simulink model "Porsche930Turbo_Model_V0"  (R2025b)
settings: Solver=ode3  StartTime=0.0  StopTime=1800  FixedStep=0.005  MaxStep=0.01  RelTol=1e-3
values from neighbouring files (symbols this model uses):
  a_front = (1 - CoG_front) * wb    (= 1.32912)    [Main.m]
  af = 1.77    [Main.m]
  bsfc = 395    [Main.m]
  cd = 0.39    [Main.m]
  crr = 0.015    [Main.m]
  distance_imola = s_track    [Main.m]
  eta_gb = 0.95    [Main.m]
  gear_numbers = [1, 2, 3, 4]    [Main.m]
  gear_ratios = [2.25, 1.30, 0.89, 0.625]    [Main.m]
  gear_shift_tbl = [1, 2, 3, 4]    [Main.m]
  grade_imola = grade_track    [Main.m]
  kt = 1.65    [Main.m]
  m_eq = mg + (J_wheels / rw^2) + (J_drivetrain * i_avg^2 / rw^2)    [Main.m]
  mg = mc + (mh * np) + mp_hybrid    (= 1492.5)    [Main.m]
  mu_road = 0.9    [Main.m]
  n_ice = 0:dn:nd    [Main.m]
  ne_em = 0:dn:nemax_em    [Main.m]
  nparallel = 2    [Main.m]
  nseries = 96    [Main.m]
  rho_fuel = 0.75    [Main.m]
  ro = 1.204    [Main.m]
  rt = 4.222    [Main.m]
  rw = (dw * 25.4 / 2 + wt * art / 100) * 1e-3    (= 0.31345)    [Main.m]
  t_ice = zeros(size(n_ice))    [Main.m]
  t_roma_san_basilio = [0 1 2 3 4 5 6 7 8 9 10 11 ... (522 elements, 522x1)]    [ECE_EUDC_Artemis_Bologna_Roma_WLTC_EE_bus.mat]
  tau_turbo = 0.6    [Main.m]
  te_em = zeros(size(ne_em))    [Main.m]
  te_em_peak = zeros(size(ne_em))    [Main.m]
  temax_em = 230    [Main.m]
  tmax_ice = 412    [Main.m]
  track_length = 4909    [Main.m]
  v_cutoff_bp = [0, 0.5, 1.4, 50]    [Main.m]
  v_cutoff_tbl = [0, 0,   1,   1 ]    [Main.m]
  v_ref_imola = v_track_ms    [Main.m]
  v_shift_bp = [0, 18, 33, 48]    [Main.m]
  v_shift_bp_EMODE = [0, 5, 22, 35]    [Main.m]
  vkm_roma_san_basilio = [28.8 30.9 32.4 34.2 35.3 35.6 34.8 33.8 32.2 30.5 29.1 27.9 ... (522 elements, 522x1)]    [ECE_EUDC_Artemis_Bologna_Roma_WLTC_EE_bus.mat]
  wb = 2.272    [Main.m]
undefined symbols (not defined in the file or in its folder): SoC_Per
libraries: simulink x58
(part 2 of 5)

== system Porsche930Turbo_Model_V0/E-MOTOR ==
  T_req_EM [Nm] : Inport
  "   " : Product
  "          " : Saturate  UpperLimit=600  LowerLimit=150
  Bus Selector3 : BusSelector  OutputSignals=trqMax,trqMin,pwrIn,pwrLoss
  Derating_LUT : Lookup_n-D  NumberOfTableDimensions=1  BreakpointsForDimension1=[20, 75, 95, 120]  Table=[2.0, 2.0, 1.0, 0.5]  InternalRulePriority=Speed  RndMeth=Simplest
  EM_model_v47b : Subsystem  mask(LEMAD Electric Drive Model v4.7.3b){pp=6, a=2.394, Linput=Lq - r, Ld_in=0.00022, Lq_in=0.000412, r_in=1, Ls_in=0.0022, sigma_in=0.9, Inn=92.93, spdIn=rpm, RsSlct=From port, overl=From Port, Rs_value=0.001, Ilim1=1.5, chk_sat=off, sat=0.2, chk_r=off, ISO=0.98, actv=From Parameters, mot_eff=95, k_cu=0.12, k_hy=0.06, k_pc=0.000003, mot_adv=off, B_mag=1.35, stray_actv=Constant Offset, stray_pct=0.4, stray_off=20, k_s2=0, k_s1=-2.12, k_s0=767, stray_watt=[100 100;100 100], stray_rpm=[0 12000], stray_vdc=[0 1000], inv_act=Constant Efficiency, inv_pwr=300, inv_eff=97, freq_slct=Fixed, f_switch=5000, tswON=0.99e-7, tswOF=0.99e-7, R_ds=7e-3, V_f=3, t_dead=10e-8, V_drv=12, Q_gTot=5e-5, R_ghi=5e-3, R_glo=2e-3, R_g=5e-3, R_gi=1e-3, k_invFix=0}
      mask prompts: pp "Pole Pairs: pp"; a "Flux coefficient: a"; Linput "Input Type"; Ld_in "Ld [H]"; Lq_in "Lq [H]"; r_in "r (Ld/Lq)"; Ls_in "Ls (H)"; sigma_in "sigma"; Inn "Rated Current: Inn [Arms]"; spdIn "Input Speed"; RsSlct "Stator Resistance"; overl "Overload"; Rs_value "Resistance value [Ohm]"; Ilim1 "PerUnit Current Overload"; chk_sat "IM saturation id min"; sat "id sat [pu]"; chk_r "Anisotropic limit"; ISO "Max admissible 'r'"; actv "Motor losses model"; mot_eff "Motor Efficiency [0-100%]:"; k_cu "k_cu : Copper losses coefficent"; k_hy "k_hy : hysteresis coefficient"; k_pc "k_pc : Parassitic Current coefficient"; mot_adv "Advanced"; B_mag "B: Magnetic remanence [T]"; stray_actv "Stray losses model"; stray_pct "Constant Percentage [0-2%]:"; stray_off "Constant stray losses [W]:"; k_s2 "k_s2: i^2 coefficient"; k_s1 "k_s1: i coefficient"; k_s0 "k_s0: offset coefficient"; stray_watt "DataMap: stray losses output [W]"; stray_rpm "DataMap: speed input [rpm]"; stray_vdc "DataMap: Vdc input [V]"; inv_act "Losses model"; inv_pwr "Inverter Power usage [W]"; inv_eff "Inverter Efficiency [0-100%]"; freq_slct "Switching Frequency"; f_switch "Frequency [Hz]:"; tswON "Switching time ON [s]:"; tswOF "Switching time OFF [s]:"; R_ds "Conduction resistance [Ohm]:"; V_f "Diode forward voltage [V]:"; t_dead "Dead time [s]:"; V_drv "Driver voltage [V]:"; Q_gTot "Gate Charge [C]:"; R_ghi "High switch Resistance R_GHi [Ohm]:"; R_glo "Low switch Resistance R_GLo [Ohm]:"; R_g "Gate resistance R_G [Ohm]:"; R_gi "Internal gate resistance R_Gi [Ohm]:"; k_invFix "Constant stray losses [W]:"
      mask help:
      | LEMAD Unified Analysis Model of Electric Machine and Drive.
      | With the setting of this few parameters, any conventional electric machine can be optimally simulated in their ideal operating condition. Overall inverter losses can also be set and modelled.
      mask init:
      | %r=Ld/Lq;
      | if Linput == 1
      |     Ld = Ld_in;
      |     Lq = Lq_in;
      |     r  = Ld/Lq;
      | elseif Linput == 2
      |     Lq = Lq_in;
      |     r  = r_in;
      |     Ld = Lq*r;
      | elseif Linput == 3
      |     Ld = Ls_in;
      |     Lq = sigma_in * Ld;
      |     r  = Ld/Lq;
      | end
      | 
      | % nominal current peak (Inn is rms)
      | In = max(0.01, (Inn*sqrt(2)));
      | 
      | % isomachine and r checks
      | if chk_r == 1
      |     ISO = min(1.05 ,max(0.94 ,ISO))
      | else
      |     ISO = 0.985;
      | end
      | if r>=ISO && r<=1+(1-ISO)
      |     Ld = Lq;
      |     r  = 1;
      | end
      | r1 = 1-(1/r);
      | r1 = max(-300 ,min(300 ,r1));
      | 
      | % IM id saturation
      | if chk_sat == 1
      |     sat = max(0.01 ,min(0.9 ,sat));   
      | else 
      |     sat = 0.01;
      | end
      | 
      | % iLim and Rs  selection
      | if overl == 2
      |     i_lim = max(0,Ilim1);
      | else
      |     i_lim = -1;
      | end
      | if RsSlct == 2
      |     rs = max(0.0001,Rs_value);
      | else
      |     rs = -1;
      | end
      | 
      | % motor losses
      | B_m = 1.35;
      | if actv==2
      |     mot_eff = min(100, max(0, mot_eff));
      |     mot_eff = mot_eff*0.01;
      | elseif actv==3
      |     stray_pct = min(5, max(0, stray_pct));
      |     stray_pct = stray_pct*0.01;
      |     stray_off = min(8e3, max(-5e3, stray_off));
      |     if B_mag >= 0.1
      |         B_m = min(3 ,max(0.1 ,B_mag));
      |     end
      | end
      | 
      | % inverter losses
      | f_sw = 1000;  t_sw = 1e-6;
      | k_driver = 1;
      | if V_drv <0;    V_drv  = 12;     end
      | if inv_act == 2; % constant power loss
      |     if inv_pwr <0
      |         inv_pwr = 100;
      |     else
      |         inv_pwr = max(0,inv_pwr);
      |     end
      | elseif inv_act == 3; % constant efficiency
      |     if inv_eff <0
      |         inv_eff = 98;
      |     else
      |         inv_eff = min(100, max(0, inv_eff));
      |         inv_eff = inv_eff*0.01;
      |     end
      | elseif inv_act == 4;   %calc from data
      |     if tswON <0;    tswON = 1e-7;   end
      |     if tswOF <0;    tswOF = 1e-7;   end
      |     t_sw = tswON + tswOF;
      |     
      |     if freq_slct==1
      |         if f_switch>0
      |             f_sw = min(1e8 ,max(1 ,f_switch));
      |         else
      |             f_sw = 8000;
      |         end
      |     else
      |         f_sw = 9;
      |     end
      |     
      |     if R_ds  <0;    R_ds   = 1e-3;   end
      |     
      |     if V_f   <0;    V_f    = 1.2;    end
      |     if t_dead<0;    t_dead = 5e-8;   end
      |     
      |     %if V_drv <0;    V_drv  = 12;     end
      |     if Q_gTot<0;    Q_gTot = 5e-5;   end
      |     if R_ghi <0;    R_ghi  = 1e-3;   end
      |     if R_glo <0;    R_glo  = 1e-3;   end
      |     if R_g   <0;    R_g    = 3e-3;   end
      |     if R_gi  <0;    R_gi   = 1e-3;   end
      |     
      |     den_hi = R_ghi+R_g+R_gi;
      |     den_lo = R_glo+R_g+R_gi;
      |     k_driver = 0.5*Q_gTot*V_drv * ((R_ghi/den_hi)+(R_glo/den_lo));
      | 
      | end %end inv_act slct
      mask Help:
      | Partial output description:
      | 
      | "id" -> D axis current [A]
      | "iq" -> Q axis current [A]
      | "iBat" -> battery current [A], positive if drive is using power from the battery
      | 
      | "trqOut" -> torque output [Nm]
      | "trqRef"-> torque reference [Nm], equal to the input "trq_ref"
      | "trqMax"-> maximum positive torque available [Nm]
      | "trqMin" -> minimum negative torque available [Nm]
      | 
      | "pwrIn"-> power input, electrical power on the input side [W]
      | "pwrOut"-> power output, mechanical power produced [W]
      | "pwrLoss"-> power losses, total (motor+inverter) [W]
      | 
      | "effTot"-> total efficiency of the system in percentage [0-1]
      mask TypeOptions Linput: Ld - Lq | Lq - r | Ls - sigma
      mask Callback Linput:
      | in   = get_param(gcb,'Linput');
      | 
      | Vis = get_param(gcb,'MaskVisibilities');
      | %Enb = get_param(gcb,'MaskEnables');
      | 
      | if     strcmpi(in,'Ld - Lq')
      |     Vis{4}  = 'on';  Vis{5}  = 'on';
      |     Vis{6}  = 'off';
      |     Vis{7}  = 'off'; Vis{8}  = 'off';
      | elseif strcmpi(in,'Lq - r')
      |     Vis{4}  = 'off'; Vis{5}  = 'on';
      |     Vis{6}  = 'on';
      |     Vis{7}  = 'off'; Vis{8}  = 'off';
      | elseif strcmpi(in,'Ls - sigma')
      |     Vis{4}  = 'off'; Vis{5}  = 'off';
      |     Vis{6}  = 'off';
      |     Vis{7}  = 'on';  Vis{8}  = 'on';
      | end
      | 
      | set_param(gcb,'MaskVisibilities',Vis);
      | 
      | clearvars Vis in;
      mask TypeOptions spdIn: rpm | rad/s
      mask TypeOptions RsSlct: None | Static | From port
      mask Callback RsSlct:
      | in   = get_param(gcb,'RsSlct');
      | 
      | Vis = get_param(gcb,'MaskVisibilities');
      | %Enb = get_param(gcb,'MaskEnables');
      | 
      | if     strcmpi(in,'Static')
      |     Vis{13}  = 'on';
      | else
      |     Vis{13}  = 'off';
      | end
      | 
      | set_param(gcb,'MaskVisibilities',Vis);
      | 
      | clearvars Vis in;
      mask TypeOptions overl: None | Static | From Port
      mask Callback overl:
      | in   = get_param(gcb,'overl');
      | 
      | Vis = get_param(gcb,'MaskVisibilities');
      | %Enb = get_param(gcb,'MaskEnables');
      | 
      | if     strcmpi(in,'Static')
      |     Vis{14}  = 'on';
      | else
      |     Vis{14}  = 'off';
      | end
      | 
      | set_param(gcb,'MaskVisibilities',Vis);
      | 
      | clearvars Vis in;
      mask Callback chk_sat:
      | in   = get_param(gcb,'chk_sat');
      | 
      | Vis = get_param(gcb,'MaskVisibilities');
      | %Enb = get_param(gcb,'MaskEnables');
      | 
      | if     strcmpi(in,'on')
      |     Vis{16}  = 'on';
      | elseif strcmpi(in,'off')
      |     Vis{16}  = 'off';
      | end
      | 
      | set_param(gcb,'MaskVisibilities',Vis);
      | %set_param(gcb,'MaskEnables',Enb);
      | clearvars Vis in;
      mask Callback chk_r:
      | in   = get_param(gcb,'chk_r');
      | 
      | Vis = get_param(gcb,'MaskVisibilities');
      | %Enb = get_param(gcb,'MaskEnables');
      | 
      | if     strcmpi(in,'on')
      |     Vis{18}  = 'on';
      | elseif strcmpi(in,'off')
      |     Vis{18}  = 'off';
      | end
      | 
      | set_param(gcb,'MaskVisibilities',Vis);
      | %set_param(gcb,'MaskEnables',Enb);
      | clearvars Vis in;
      mask TypeOptions actv: Ideal | Fixed Efficiency | From Parameters
      mask Callback actv:
      | in   = get_param(gcb,'actv');
      | 
      | ina   = get_param(gcb,'mot_adv');
      | inb   = get_param(gcb,'stray_actv');
      | 
      | Vis = get_param(gcb,'MaskVisibilities');
      | %Enb = get_param(gcb,'MaskEnables');
      | 
      | rng = [20 21 22 23 25 27 28 29 30 31 32 33 34];
      | for kk=1:length(rng)
      |     Vis{rng(kk)} = 'off';
      | end
      | 
      | if     strcmpi(in,'Ideal')
      |     Vis{20}  = 'off'; Vis{24} = 'off'; Vis{26} = 'off';
      | elseif strcmpi(in,'Fixed Efficiency')
      |     Vis{20}  = 'on'; Vis{24} = 'off'; Vis{26} = 'off';
      | elseif strcmpi(in,'From Parameters')
      |     Vis{21}  = 'on'; Vis{22}  = 'on'; Vis{23}  = 'on'; Vis{24}  = 'on';
      |     if     strcmpi(ina,'on')
      |         Vis{25}  = 'on'; Vis{26}  = 'on';
      |         if     strcmpi(inb,'Constant Percentage')
      |             Vis{27}  = 'on';
      |         elseif strcmpi(inb,'Constant Offset')
      |             Vis{28}  = 'on';
      |         elseif strcmpi(inb,'Generic Polynom')
      |             Vis{29}  = 'on'; Vis{30}  = 'on'; Vis{31}  = 'on';
      |         elseif strcmpi(inb,'From Data Map')
      |             Vis{32}  = 'on'; Vis{33}  = 'on'; Vis{34}  = 'on';
      |         end
      |     else
      |         Vis{25}  = 'off'; Vis{26} = 'off';
      |     end
      | end
      | 
      | set_param(gcb,'MaskVisibilities',Vis);
      | 
      | clearvars Vis in ina inb rng kk;
      mask Callback mot_adv:
      | in   = get_param(gcb,'mot_adv');
      | 
      | inb  = get_param(gcb,'stray_actv');
      | 
      | Vis = get_param(gcb,'MaskVisibilities');
      | %Enb = get_param(gcb,'MaskEnables');
      | 
      | rng = [25 27 28 29 30 31 32 33 34];
      | for kk=1:length(rng)
      |     Vis{rng(kk)} = 'off';
      | end
      | 
      | if     strcmpi(in,'on')
      |     Vis{25}  = 'on'; Vis{26}  = 'on';
      |     if     strcmpi(inb,'Constant Percentage')
      |         Vis{27}  = 'on';
      |     elseif strcmpi(inb,'Constant Offset')
      |         Vis{28}  = 'on';
      |     elseif strcmpi(inb,'Generic Polynom')
      |         Vis{29}  = 'on'; Vis{30}  = 'on'; Vis{31}  = 'on';
      |     elseif strcmpi(inb,'From Data Map')
      |         Vis{32}  = 'on'; Vis{33}  = 'on'; Vis{34}  = 'on';
      |     end
      | else
      |     Vis{25}  = 'off'; Vis{26}  = 'off';
      | end
      | 
      | set_param(gcb,'MaskVisibilities',Vis);
      | 
      | clearvars Vis in inb rng kk;
      mask TypeOptions stray_actv: None | Constant Percentage | Constant Offset | Generic Polynom | From Data Map
      mask Callback stray_actv:
      | in   = get_param(gcb,'stray_actv');
      | 
      | Vis = get_param(gcb,'MaskVisibilities');
      | %Enb = get_param(gcb,'MaskEnables');
      | 
      | rng = 27:34;
      | for kk=1:length(rng)
      |     Vis{rng(kk)} = 'off';
      | end
      | 
      | if     strcmpi(in,'Constant Percentage')
      |     Vis{27}  = 'on';
      | elseif strcmpi(in,'Constant Offset')
      |     Vis{28}  = 'on';
      | elseif strcmpi(in,'Generic Polynom')
      |     Vis{29}  = 'on'; Vis{30}  = 'on'; Vis{31}  = 'on';
      | elseif strcmpi(in,'From Data Map')
      |     Vis{32}  = 'on'; Vis{33}  = 'on'; Vis{34}  = 'on';
      | end
      | 
      | set_param(gcb,'MaskVisibilities',Vis);
      | 
      | clearvars Vis in rng kk;
      mask TypeOptions inv_act: Ideal Inverter | Constant Losses | Constant Efficiency | Advanced Losses
      mask Callback inv_act:
      | in   = get_param(gcb,'inv_act');
      | 
      | Vis = get_param(gcb,'MaskVisibilities');
      | %Enb = get_param(gcb,'MaskEnables');
      | 
      | rng = 36:51;
      | for kk=1:length(rng)
      |     Vis{rng(kk)} = 'off';
      | end
      | 
      | if     strcmpi(in,'Constant Losses')
      |     Vis{36}  = 'on';
      | elseif strcmpi(in,'Constant Efficiency')
      |     Vis{37}  = 'on';
      | elseif strcmpi(in,'Advanced Losses')
      |     Vis{38}  = 'on';
      |     %Vis{39}  = 'on';
      |     Vis{40}  = 'on';  Vis{41}  = 'on';
      |     Vis{42}  = 'on';  Vis{43}  = 'on'; Vis{44}  = 'on';
      |     Vis{45}  = 'on';  Vis{46}  = 'on'; Vis{47}  = 'on';
      |     Vis{48}  = 'on';  Vis{49}  = 'on'; Vis{50}  = 'on'; Vis{51}  = 'on';
      |     in2   = get_param(gcb,'freq_slct');
      |     if strcmpi(in2,'Variable')
      |          Vis{39}  = 'off';
      |     else %if strcmpi(in2,'Variable')
      |          Vis{39}  = 'on';
      |     end
      | end
      | 
      | set_param(gcb,'MaskVisibilities',Vis);
      | 
      | clearvars Vis in in2 rng kk;
      mask TypeOptions freq_slct: Fixed | Variable
      mask Callback freq_slct:
      | in   = get_param(gcb,'freq_slct');
      | 
      | Vis = get_param(gcb,'MaskVisibilities');
      | %Enb = get_param(gcb,'MaskEnables');
      | 
      | if     strcmpi(in,'Fixed')
      |     Vis{39}  = 'on';
      | elseif strcmpi(in,'Variable')
      |     Vis{39}  = 'off';
      | end
      | 
      | set_param(gcb,'MaskVisibilities',Vis);
      | 
      | clearvars Vis in;
      mask DialogControl Container11 Prompt: Inductance Parameters Input
      mask DialogControl Container6 Prompt: Advanced Settings
      mask DialogControl Container14 Prompt: Motor Losses
      mask DialogControl Control4 Prompt: The parameter model function performes the analytical calculation of the electrical losses of the electric motor using the formula:
      mask DialogControl Control5 Prompt: P = k_cu * I^2 + k_i*w*B^2.2 + k_cp*w^2*B^2
      mask DialogControl Control6 Prompt: where w is the stator frequency.
      mask DialogControl Container13 Prompt: Inverter Losses
      mask DialogControl Control8 Prompt: Leave "-1" for standard value.
      mask DialogControl Container15 Prompt: Switching Losses
      mask DialogControl Container18 Prompt: Conduction Losses
      mask DialogControl Container17 Prompt: Diode Losses
      mask DialogControl Container16 Prompt: Driver Circuit Losses
      mask DialogControl Container20 Prompt: Stray Losses
      mask Display:
      | fprintf('EM Drive\nLEMAD U.A.')
      | % Inports
      | port_label('input', 1, 'trq_ref [Nm]')
      | if spdIn == 1
      |     port_label('input', 2, 'spd [rpm]')
      | else
      |     port_label('input', 2, 'spd [rad/s]')
      | end
      | port_label('input', 3, 'Vdc [V]')
      | if overl == 3
      |     port_label('input', 4, 'I_lim [pu]')
      | else
      |     port_label('input', 4, '~')
      | end
      | if RsSlct == 3
      |     port_label('input', 5, 'Rs [Ohm]')
      | else
      |     port_label('input', 5, '~')
      | end
      | if (inv_act==4 && freq_slct == 2)
      |     port_label('input', 6, 'SwitchFreq [Hz]')
      | else
      |     port_label('input', 6, '~')
      | end
      | 
      | % {
      | % Outports
      | port_label('output', 1, 'outBus')
      | %}
      | %{
      | % Outports
      | port_label('output', 1, 'idq')
      | port_label('output', 2, 'I_bat')
      | port_label('output', 3, 'trq')
      | port_label('output', 4, 'pwr')
      | port_label('output', 5, 'eff')
      | %}
  Rs : Constant  Value=0.015
  Sat_EM_torque : simulink/Discontinuities/Saturation Dynamic  OutMin=[]  OutMax=[]  OutDataTypeStr=Inherit: Same as second input  OutDataType=fixdt(1, 16)  OutScaling=2^-10  DoSatur=off
  Thermal_Management : Subsystem
  fsw : Constant  Value=8000
  rpm : Gain  Gain=rt * 60 / (2 * pi * rw)
  T_EM_real [Nm] : Outport
  P_batt [W] : Outport  Port=2
  Temp_EM [°C] : Outport  Port=3
  wires:
  [speed] -> "   "/1
  [gear_ratio] -> "   "/2
  "   "/1 -> rpm/1
  [DC_voltage] -> "          "/1
  Thermal_Management/1(Temp_EM) -> Derating_LUT/1, Temp_EM [°C]/1
  rpm/1 -> EM_model_v47b/2(spd)
  "          "/1 -> EM_model_v47b/3(Vdc [V])
  Derating_LUT/1 -> EM_model_v47b/4(I_lim [pu])
  Rs/1 -> EM_model_v47b/5(Rs [Ohm])
  fsw/1 -> EM_model_v47b/6(swFreq[Hz])
  EM_model_v47b/1(outBus) -> Bus Selector3/1
  Bus Selector3/1 -> Sat_EM_torque/1  "<trqMax>"
  Bus Selector3/2 -> Sat_EM_torque/3  "<trqMin>"
  Sat_EM_torque/1 -> T_EM_real [Nm]/1
  Bus Selector3/3 -> P_batt [W]/1  "<pwrIn>"
  Bus Selector3/4 -> Thermal_Management/1(pwrLoss)  "<pwrLoss>"
  T_req_EM [Nm]/1 -> Sat_EM_torque/2, EM_model_v47b/1(trq_ref [Nm])

== system Porsche930Turbo_Model_V0/ECU ==
  F_tract_req [N] : Inport
  speed [m/s] : Inport  Port=2
  DC voltage [V] : Inport  Port=3
  Gear : Inport  Port=4
  BatteryTemp_Derating_LUT : Lookup_n-D  NumberOfTableDimensions=1  BreakpointsForDimension1=[20, 45, 55, 60]  Table=[1.0, 1.0, 0.5, 0.0]  InternalRulePriority=Speed  RndMeth=Simplest
  Constant : Constant  Value=rw
  Constant1 : Constant  Value=rt
  Demux : Demux  Outputs=2
  Divide : Product  Inputs=*/
  Divide1 : Product  Inputs=/*
  E_Mode : Subsystem
  Gain : Gain  Gain=rw
  Gain1 : Gain  Gain=rt
  Gear ratios : Lookup_n-D  NumberOfTableDimensions=1  BreakpointsForDimension1=gear_numbers  Table=gear_ratios  InterpMethod=Flat  InternalRulePriority=Speed  RndMeth=Simplest
  Hybrid_Mode : Subsystem
  ICE_Mode : Subsystem
  Mem_EM : Memory  InheritSampleTime=on
  Mem_ICE : Memory  InheritSampleTime=on
  Mode : Constant  Value=3
  Multiport Switch : MultiPortSwitch  Inputs=4  SaturateOnIntegerOverflow=off  InputSameDT=off
  Product : Product  Inputs=3
  Product1 : Product  Inputs=3
  RACE_Mode : Subsystem
  SoC_Derating_LUT : Lookup_n-D  NumberOfTableDimensions=1  BreakpointsForDimension1=[0, 0.05, 0.20, 1.0]  Table=[0, 0, 1.0, 1.0]  InternalRulePriority=Speed  RndMeth=Simplest
  T_ICE [Nm] : Outport
  T_EM [Nm] : Outport  Port=2
  tag scope: Mode=global, T_req=global, gear_ratio=global
  wires:
  Multiport Switch/1 -> Demux/1
  Demux/1 -> Mem_ICE/1
  Mode/1 -> [Mode], Multiport Switch/1
  F_tract_req [N]/1 -> Gain/1
  Gear/1 -> Gear ratios/1
  Gear ratios/1 -> Product1/3, [gear_ratio], Gain1/1
  Gain/1 -> Divide1/2  "Wheel torque"
  Product1/1 -> Divide/1
  speed [m/s]/1 -> Product1/1
  Constant/1 -> Divide/2
  Divide/1 -> Hybrid_Mode/2(Crankshaft_speed), RACE_Mode/2(Crankshaft_speed), E_Mode/2(Crankshaft_speed)
  E_Mode/1(T_actual) -> Multiport Switch/3
  RACE_Mode/1(T_actual) -> Multiport Switch/5
  Hybrid_Mode/1(T_actual) -> Multiport Switch/4
  DC voltage [V]/1 -> E_Mode/3(DC_Voltage)
  Gain1/1 -> Divide1/1
  Constant1/1 -> Product1/2
  [Temp_Batt] -> BatteryTemp_Derating_LUT/1
  Demux/2 -> Product/1
  BatteryTemp_Derating_LUT/1 -> Product/2
  [SoC] -> SoC_Derating_LUT/1
  SoC_Derating_LUT/1 -> Product/3
  Product/1 -> Mem_EM/1
  Mem_EM/1 -> T_EM [Nm]/1
  Mem_ICE/1 -> T_ICE [Nm]/1
  ICE_Mode/1(T_actual) -> Multiport Switch/2  "T_ICE"
  Divide1/1 -> [T_req], ICE_Mode/1(T_req), RACE_Mode/1(T_req), Hybrid_Mode/1(T_req), E_Mode/1(T_req)  "PWT_Torque"
  [SoC] -> Hybrid_Mode/3(SoC), RACE_Mode/3(SoC)

== system Porsche930Turbo_Model_V0/Gear Shifter ==
  Compare To Constant : simulink/Logic and Bit Operations/Compare To Constant  relop===  const=2  OutDataTypeStr=boolean
  Gear Shifter : Lookup_n-D  NumberOfTableDimensions=1  BreakpointsForDimension1=v_shift_bp  Table=gear_shift_tbl  InterpMethod=Flat  InternalRulePriority=Speed  RndMeth=Simplest
  Gear Shifter E-Mode : Lookup_n-D  NumberOfTableDimensions=1  BreakpointsForDimension1=v_shift_bp_EMODE  Table=gear_shift_tbl  InterpMethod=Flat  InternalRulePriority=Speed  RndMeth=Simplest
  Switch : Switch  Criteria=u2 > Threshold  SaturateOnIntegerOverflow=off  InputSameDT=off
  Gear : Outport
  wires:
  [speed] -> Gear Shifter/1
  [speed] -> Gear Shifter E-Mode/1
  Gear Shifter E-Mode/1 -> Switch/1
  [Mode] -> Compare To Constant/1
  Gear Shifter/1 -> Switch/3
  Compare To Constant/1 -> Switch/2
  Switch/1 -> Gear/1

== system Porsche930Turbo_Model_V0/Gearbox ==
  T_in [Nm] : Inport
  Gear : Inport  Port=2
  1-D Lookup Table : Lookup_n-D  NumberOfTableDimensions=1  BreakpointsForDimension1=gear_numbers  Table=gear_ratios  InterpMethod=Flat  InternalRulePriority=Speed  RndMeth=Simplest
  Gain : Gain  Gain=rt * eta_gb / rw
  Product : Product
  F_trac_real [N] : Outport
  tag scope: F_traction=global
  wires:
  Gear/1 -> 1-D Lookup Table/1
  1-D Lookup Table/1 -> Product/2
  T_in [Nm]/1 -> Product/1
  Product/1 -> Gain/1
  Gain/1 -> [F_traction], F_trac_real [N]/1

== system Porsche930Turbo_Model_V0/ICE ==
  T_ICE_req [Nm] : Inport
  1-D Lookup Table : Lookup_n-D  NumberOfTableDimensions=1  BreakpointsForDimension1=n_ice  Table=t_ice  ExtrapMethod=Clip  InternalRulePriority=Speed  RndMeth=Simplest
  Constant : Constant  Value=0
  Gain : Gain  Gain=rt * 60 / (2 * pi * rw)
  ICE energy consumption : Subsystem
  Product : Product
  Saturation Dynamic : simulink/Discontinuities/Saturation Dynamic  OutMin=[]  OutMax=[]  OutDataTypeStr=Inherit: Same as second input  OutDataType=fixdt(1, 16)  OutScaling=2^-10  DoSatur=off
  Scope : Scope  NumInputPorts=4
      settings: ActiveDisplayYMinimum=-1  ActiveDisplayYMaximum=1  DataLoggingVariableName=ScopeData26
  Transfer Fcn : TransferFcn  Denominator=[tau_turbo 1]
  T_ICE_real [Nm] : Outport
  P_ICE [W] : Outport  Port=2
  wires:
  [speed] -> Product/1
  [gear_ratio] -> Product/2
  Product/1 -> Gain/1
  T_ICE_req [Nm]/1 -> Scope/2, Transfer Fcn/1
  Gain/1 -> ICE energy consumption/1(RPM), 1-D Lookup Table/1  "RPM"
  Transfer Fcn/1 -> Scope/3, Saturation Dynamic/2
  1-D Lookup Table/1 -> Saturation Dynamic/1, Scope/4
  Constant/1 -> Saturation Dynamic/3
  Saturation Dynamic/1 -> Scope/1, T_ICE_real [Nm]/1, ICE energy consumption/2(T_ICE)
  ICE energy consumption/1(P_ICE [W]) -> P_ICE [W]/1

== system Porsche930Turbo_Model_V0/Lap TIme ==
  distance [m] : Inport
  Clock : Clock
  Constant : Constant  Value=track_length
  MATLAB Function : MATLAB Function  TreatAsAtomicUnit=on
  Zero-Order Hold : ZeroOrderHold  SampleTime=0.01
  Zero-Order Hold1 : ZeroOrderHold  SampleTime=0.01
  lap_time_str : Outport
  lap_time_sec : Outport  Port=2
  wires:
  Clock/1 -> Zero-Order Hold/1
  distance [m]/1 -> Zero-Order Hold1/1
  Zero-Order Hold/1 -> MATLAB Function/1(t)
  Zero-Order Hold1/1 -> MATLAB Function/2(dist)
  Constant/1 -> MATLAB Function/3(L_track)
  MATLAB Function/1(lap_time_str) -> lap_time_str/1
  MATLAB Function/2(lap_time_sec) -> lap_time_sec/1

== system Porsche930Turbo_Model_V0/reference Speed  [kph] ==
  note: %%-----------------------------------------------------%%
      | %%--- Author: 	MTB 				 ---%%
      | %%--- Copyright: 	2017/18 Lemad-UniBo ---%%
      | %%--- Version:	1.2 (03/05/18)		 ---%%
      | %%-----------------------------------------------------%%
  1) Ref: urban ECE 15 - 195s : simulink/Sources/Repeating Sequence  rep_seq_t=[0 11 15 23 28 49 55 61 85 96 117 123 134 143 155 163 178 188 195]  rep_seq_y=[0 0 15 15 0 0 15 15 32 32 0 0 15 35 50 50 35 35 0]
  10) Ref: WLTC class1 - 1612s : simulink/Sources/Repeating Sequence  rep_seq_t=t_wltc_class_1  rep_seq_y=vkm_wltc_class_1
  11) Ref: WLTC class2 - 1800s : simulink/Sources/Repeating Sequence  rep_seq_t=t_wltc_class_2  rep_seq_y=vkm_wltc_class_2
  12) Ref: WLTC class3a - 1800s : simulink/Sources/Repeating Sequence  rep_seq_t=t_wltc_class_3a  rep_seq_y=vkm_wltc_class_3a
  13) Ref: WLTC class3b - 1800s : simulink/Sources/Repeating Sequence  rep_seq_t=t_wltc_class_3b  rep_seq_y=vkm_wltc_class_3b
  14) Ref: Bus line BO 27A - 3246s : simulink/Sources/Repeating Sequence  rep_seq_t=t_bus_27A  rep_seq_y=vkm_bus_27A
  15) Ref: Bus line BO 27B - 3058s : simulink/Sources/Repeating Sequence  rep_seq_t=t_bus_27B  rep_seq_y=vkm_bus_27B
  16) Ref: Bus line BO 33 - 1850s : simulink/Sources/Repeating Sequence  rep_seq_t=t_bus_33  rep_seq_y=vkm_bus_33
  17) Ref: EE Bike Cycle - 1201s : simulink/Sources/Repeating Sequence  rep_seq_t=EE_time  rep_seq_y=EE_Speedkmh
  2) Ref: Rural EUDC - 400s : simulink/Sources/Repeating Sequence  rep_seq_t=t_eudc  rep_seq_y=vkm_eudc
  3) Ref: Artemis urban- 994s : simulink/Sources/Repeating Sequence  rep_seq_t=t_artemis_urban  rep_seq_y=vkm_artemis_urban
  4) Ref: Artemis rural - 1083s : simulink/Sources/Repeating Sequence  rep_seq_t=t_artemis_rural  rep_seq_y=vkm_artemis_rural
  5) Ref: Artemis motorway - 1068s : simulink/Sources/Repeating Sequence  rep_seq_t=t_artemis_motorway130  rep_seq_y=vkm_artemis_motorway130
  6) Ref: Roma S. Basilio - 522s : simulink/Sources/Repeating Sequence  rep_seq_t=[-0.1 ; t_roma_san_basilio]  rep_seq_y=[0 ; vkm_roma_san_basilio]
  7) Ref: Viali Bologna LENTO - 1321s : simulink/Sources/Repeating Sequence  rep_seq_t=t_bologna_viali_lento  rep_seq_y=vkm_bologna_viali_lento
  8) Ref: Viali Bologna VELOCE - 1215s : simulink/Sources/Repeating Sequence  rep_seq_t=t_bologna_viali_veloce  rep_seq_y=vkm_bologna_viali_veloce
  9) Ref: WLTC city - 1022s : simulink/Sources/Repeating Sequence  rep_seq_t=t_wltc_city  rep_seq_y=vkm_wltc_city
  Index Vector : MultiPortSwitch  Inputs=18  SaturateOnIntegerOverflow=off  InputSameDT=off
  Smoo : RateLimiter  RisingSlewLimit=9  FallingSlewLimit=-9  SampleTimeMode=inherited
  max : Constant  Value=130
  select cycle : Constant  Value=slct
  v_kph : Outport
  wires:
  max/1 -> Index Vector/19
  17) Ref: EE Bike Cycle - 1201s/1 -> Index Vector/18
  16) Ref: Bus line BO 33 - 1850s/1 -> Index Vector/17
  15) Ref: Bus line BO 27B - 3058s/1 -> Index Vector/16
  14) Ref: Bus line BO 27A - 3246s/1 -> Index Vector/15
  select cycle/1 -> Index Vector/1
  2) Ref: Rural EUDC - 400s/1 -> Index Vector/3
  3) Ref: Artemis urban- 994s/1 -> Index Vector/4
  4) Ref: Artemis rural - 1083s/1 -> Index Vector/5
  5) Ref: Artemis motorway - 1068s/1 -> Index Vector/6
  Smoo/1 -> Index Vector/7
  7) Ref: Viali Bologna LENTO - 1321s/1 -> Index Vector/8
  8) Ref: Viali Bologna VELOCE - 1215s/1 -> Index Vector/9
  9) Ref: WLTC city - 1022s/1 -> Index Vector/10
  10) Ref: WLTC class1 - 1612s/1 -> Index Vector/11
  11) Ref: WLTC class2 - 1800s/1 -> Index Vector/12
  12) Ref: WLTC class3a - 1800s/1 -> Index Vector/13
  13) Ref: WLTC class3b - 1800s/1 -> Index Vector/14
  Index Vector/1 -> v_kph/1
  6) Ref: Roma S. Basilio - 522s/1 -> Smoo/1
  1) Ref: urban ECE 15 - 195s/1 -> Index Vector/2

== system Porsche930Turbo_Model_V0/vehicle dynamics ==
  F_MOT [N] : Inport
  F_brake_mech [N] : Inport  Port=2
  " " : Gain  Gain=mu_road
  F_acc : Sum  Inputs=-++
  Fz_rear_static : Constant  Value=mg * 9.81 * (a_front / wb)
  GreaterThan : RelationalOperator  Operator=>  OutDataTypeStr=boolean  RndMeth=Simplest  InputSameDT=off
  Imola Grade [pu] : Lookup_n-D  NumberOfTableDimensions=1  BreakpointsForDimension1=distance_imola  Table=grade_imola  InternalRulePriority=Speed  RndMeth=Simplest
  Imola racetrack length [m] : Constant  Value=4909
  Integrator : Integrator  LimitOutput=on  LowerSaturationLimit=0
  Manual Switch : ManualSwitch
  Manual Switch1 : ManualSwitch  CurrentSetting=0
  Memory : Memory
  Scope : Scope  NumInputPorts=3
      settings: ActiveDisplayYMinimum=-9635.887828125  ActiveDisplayYMaximum=9635.887828125  DataLoggingVariableName=ScopeData28
  Scope1 : Scope
      settings: ActiveDisplayYMinimum=-1  ActiveDisplayYMaximum=1  DataLoggingVariableName=ScopeData33
  Scope2 : Scope
      settings: ActiveDisplayYMinimum=-1  ActiveDisplayYMaximum=1  DataLoggingVariableName=ScopeData35
  Scope3 : Scope
      settings: ActiveDisplayYMinimum=-1  ActiveDisplayYMaximum=1  DataLoggingVariableName=ScopeData42
  Stop Simulation : Stop
  Traction_Sat : simulink/Discontinuities/Saturation Dynamic  OutMin=[]  OutMax=[]  OutDataTypeStr=Inherit: Same as second input  OutDataType=fixdt(1, 16)  OutScaling=2^-10  DoSatur=off
  "acceleration " : Gain  Gain=1/m_eq
  grade [pu] : Constant  Value=0
  max braking force : Gain  Gain=-1
  vehicle load forces : Subsystem
  speed : Outport
  tag scope: F_LOAD=global
  wires:
  Fz_rear_static/1 -> " "/1
  " "/1 -> Scope/1, Traction_Sat/1, max braking force/1  "max traction force"
  F_MOT [N]/1 -> Scope/2, Traction_Sat/2
  max braking force/1 -> Scope/3, Traction_Sat/3
  F_acc/1 -> "acceleration "/1
  Integrator/1 -> Memory/1
  Traction_Sat/1 -> F_acc/2
  [F_LOAD] -> F_acc/1
  Manual Switch/1 -> vehicle load forces/1(road grade)
  grade [pu]/1 -> Manual Switch/1
  [distance_m] -> GreaterThan/1, Imola Grade [pu]/1
  Imola racetrack length [m]/1 -> GreaterThan/2
  Imola Grade [pu]/1 -> Manual Switch/2
  F_brake_mech [N]/1 -> F_acc/3
  Memory/1 -> vehicle load forces/2(speed [m/s]), Scope1/1, speed/1
  vehicle load forces/1(F_LOAD [N]) -> Scope2/1, [F_LOAD]
  Manual Switch1/1 -> Stop Simulation/1
  GreaterThan/1 -> Manual Switch1/1
  "acceleration "/1 -> Integrator/1, Scope3/1

== system Porsche930Turbo_Model_V0/Battery Pack/Subsystem ==
  note: %%-----------------------------------------------------%%
      | %%--- Author: 	CF 					 ---%%
      | %%--- Copyright: 	2019-21 Lemad-UniBo ---%%
      | %%--- Version:	0.3.2 (25/05/21)		 ---%%
      | %%-----------------------------------------------------%%
  iB [A] : Inport
  TAmb [°C] : Inport  Port=2
  BMS : Subsystem
  Constant : Constant  Value=0  OutDataTypeStr=single
  Data Type Conversion : DataTypeConversion  OutDataTypeStr=single  SaturateOnIntegerOverflow=off  RndMeth=Floor
  Data Type Conversion1 : DataTypeConversion  OutDataTypeStr=single  SaturateOnIntegerOverflow=off  RndMeth=Floor
  Delay1 : Delay  DelayLength=1
  Gain : Gain  Gain=1/parallelNumber  OutDataTypeStr=single
  Gain1 : Gain  Gain=seriesNumber
  SOC Evalutation : Subsystem
      mask Display: image('SOC.PNG'); % Use "Edit Image" on toolstrip to change.
  SOH [%] : Constant  Value=InitialSOH  OutDataTypeStr=single
  Scope : Scope
      settings: ActiveDisplayYMinimum=-1  ActiveDisplayYMaximum=1  DataLoggingSaveFormat=Array
  Scope1 : Scope  NumInputPorts=3
      settings: ActiveDisplayYMinimum=338.29637145996094  ActiveDisplayYMaximum=391.70899963378906  DataLoggingVariableName=ScopeData2  DataLoggingSaveFormat=Array
  Stop Simulation : Stop
  Switch : Switch  Threshold=1  SaturateOnIntegerOverflow=off  InputSameDT=off
  Thermal Model : Subsystem
      mask Display: image('ThermModel.png'); % Use "Edit Image" on toolstrip to change.
  Vb Evaluation : Subsystem
      mask Display: image('SP_scheme.PNG'); % Use "Edit Image" on toolstrip to change.
  vB [V] : Outport
  CellT [°C] : Outport  Port=2
  SOC [%] : Outport  Port=3
  PowrLoss(t) [W] : Outport  Port=4
  wires:
  SOH [%]/1 -> Vb Evaluation/3(SOH [%]), SOC Evalutation/2(SOH [%])
  SOC Evalutation/1(SOC [%]) -> Scope/1, SOC [%]/1, Vb Evaluation/2(SOC [%])
  TAmb [°C]/1 -> Data Type Conversion/1
  Gain/1 -> SOC Evalutation/1(iB [A]), Scope1/2, BMS/2(iB [A]), Vb Evaluation/1(iB(t) [A])  "Cell Current [A]"
  Vb Evaluation/1(vB(t) [V]) -> Gain1/1, BMS/1(vB(t) [V])
  Gain1/1 -> Scope1/1, vB [V]/1  "Cell Voltage [V]"
  Vb Evaluation/2(PowrLoss(t) [W]) -> PowrLoss(t) [W]/1, Thermal Model/1(PowrLoss(t) [W])
  Thermal Model/1(CellT [°C]) -> BMS/3(CellT [°C]), Vb Evaluation/4(TCell [°C]), Scope1/3, CellT [°C]/1  "Cell Temperature [°C]"
  BMS/1(StopCondition) -> Stop Simulation/1
  Switch/1 -> Gain/1
  iB [A]/1 -> Data Type Conversion1/1
  Constant/1 -> Switch/1
  Delay1/1 -> Switch/2
  [StopCondition] -> Delay1/1
  Data Type Conversion/1 -> Thermal Model/2(TAmb [°C])
  Data Type Conversion1/1 -> Switch/3

== system Porsche930Turbo_Model_V0/E-MOTOR/EM_model_v47b ==
  note: %%-----------------------------------------------------%%
      | %%--- Author: 	MTB - Ivan Petrarca	 ---%%
      | %%--- Copyright: 	2017-22 Lemad            ---%%
      | %%--- Version:	4.7.3b (05/05/22)		 ---%%
      | %%-----------------------------------------------------%%
  trq_ref [Nm] : Inport
  spd : Inport  Port=2
  Vdc [V] : Inport  Port=3
  I_lim [pu] : Inport  Port=4
  Rs [Ohm] : Inport  Port=5
  swFreq[Hz] : Inport  Port=6
  Add : Sum
  Demux : Demux  Outputs=2
  Display : Display
  Imot : Sqrt
  Motor_Model : Subsystem
  Mux : Mux  Inputs=3
  Product : Product
  Product1 : Product
  pu_to_real & losses : Subsystem
  real_to_pu & param : Subsystem
  sc11 : Scope  NumInputPorts=4
      settings: Title=TORQUE  ActiveDisplayYMinimum=-280.07449559965693  ActiveDisplayYMaximum=220.6704603969124  DataLoggingVariableName=ScopeData4  DataLoggingSaveFormat=Array
  outBus : Outport
  wires:
  Motor_Model/2(trq) -> pu_to_real & losses/2(trq_pu)
  real_to_pu & param/5(c) -> Motor_Model/5(c)
  real_to_pu & param/7(T0) -> pu_to_real & losses/4(T0)
  real_to_pu & param/6(theta) -> Motor_Model/6(theta)
  Vdc [V]/1 -> [vdc], real_to_pu & param/3(Vdc)
  I_lim [pu]/1 -> real_to_pu & param/4(iLim)
  spd/1 -> real_to_pu & param/2(spd)
  trq_ref [Nm]/1 -> real_to_pu & param/1(trq)
  real_to_pu & param/3(t) -> Motor_Model/3(t)
  Motor_Model/1(idq_out) -> pu_to_real & losses/1(idq_pu)
  [vdc] -> pu_to_real & losses/3(Vdc)
  real_to_pu & param/2("b ") -> Motor_Model/2(b)
  real_to_pu & param/4(I0) -> Motor_Model/4(I0)
  real_to_pu & param/8(w_m) -> pu_to_real & losses/5(w_m)
  real_to_pu & param/1(trq_ctrl0) -> Motor_Model/1(trq_ctrl0)
  swFreq[Hz]/1 -> pu_to_real & losses/7(swFreq)
  pu_to_real & losses/6(oBus) -> outBus/1
  pu_to_real & losses/1(trq) -> sc11/1
  pu_to_real & losses/2(idq) -> Demux/1
  pu_to_real & losses/3(pwr) -> sc11/3
  pu_to_real & losses/4(iBat) -> sc11/4
  Rs [Ohm]/1 -> real_to_pu & param/5(rs_)
  real_to_pu & param/9(rs) -> pu_to_real & losses/6(rs)
  pu_to_real & losses/5(eff) -> Display/1
  Demux/1 -> Mux/1, Product/1, Product/2
  Demux/2 -> Product1/2, Mux/2, Product1/1
  Product/1 -> Add/1
  Product1/1 -> Add/2
  Add/1 -> Imot/1
  Imot/1 -> Mux/3
  Mux/1 -> sc11/2

== system Porsche930Turbo_Model_V0/E-MOTOR/Thermal_Management ==
  pwrLoss : Inport
  " " : Sum  Inputs=+-
  "  " : Sum  Inputs=|+-
  "   " : Integrator  InitialCondition=25
  Cth : Gain  Gain=1/5625
  T_ambient : Constant  Value=25
  hA : Gain  Gain=25
  Temp_EM : Outport
  wires:
  pwrLoss/1 -> "  "/1
  "  "/1 -> Cth/1
  Cth/1 -> "   "/1
  "   "/1 -> Temp_EM/1, " "/1
  T_ambient/1 -> " "/2
  " "/1 -> hA/1
  hA/1 -> "  "/2

== system Porsche930Turbo_Model_V0/ECU/E_Mode ==
  T_req : Inport
  Crankshaft_speed : Inport  Port=2
  DC_Voltage : Inport  Port=3
  1-D Lookup Table : Lookup_n-D  NumberOfTableDimensions=1  BreakpointsForDimension1=v_cutoff_bp  Table=-temax_em * v_cutoff_tbl  InternalRulePriority=Speed  RndMeth=Simplest
  Compare To Constant : simulink/Logic and Bit Operations/Compare To Constant  relop=<=  const=0.15  OutDataTypeStr=boolean
  Compare To Constant1 : simulink/Logic and Bit Operations/Compare To Constant  relop=<=  const=0.15  OutDataTypeStr=boolean
  Constant : Constant  Value=kt
  Constant1 : Constant  Value=0
  Constant3 : Constant  Value=0
  Constant4 : Constant  Value=0
  Constant5 : Constant  Value=temax_em
  GreaterThan : RelationalOperator  Operator=>  OutDataTypeStr=boolean  RndMeth=Simplest  InputSameDT=off
  Mux : Mux  Inputs=2
  Product : Product
  Saturation : Saturate  UpperLimit=inf  LowerLimit=0
  Saturation Dynamic : simulink/Discontinuities/Saturation Dynamic  OutMin=[]  OutMax=[]  OutDataTypeStr=Inherit: Same as second input  OutDataType=fixdt(1, 16)  OutScaling=2^-10  DoSatur=off
  Switch : Switch  Criteria=u2 > Threshold  SaturateOnIntegerOverflow=off  InputSameDT=off
  Switch1 : Switch  Criteria=u2 > Threshold  SaturateOnIntegerOverflow=off  InputSameDT=off
  Switch2 : Switch  Criteria=u2 > Threshold  SaturateOnIntegerOverflow=off  InputSameDT=off
  T_req1 : InportShadow
  T_actual : Outport
  wires:
  Constant/1 -> Product/1
  Product/1 -> GreaterThan/1  "BEMF"
  DC_Voltage/1 -> GreaterThan/2
  GreaterThan/1 -> Switch/2
  Constant1/1 -> Switch/1
  Mux/1 -> T_actual/1
  Saturation Dynamic/1 -> Switch2/3  "T_EMOT"
  [SoC] -> Compare To Constant/1
  Switch1/1 -> Saturation/1
  Compare To Constant/1 -> Switch1/2
  T_req1/1 -> Switch1/1
  Constant3/1 -> Switch1/3
  Compare To Constant1/1 -> Switch2/2
  [SoC] -> Compare To Constant1/1
  Constant4/1 -> Switch2/1
  Switch2/1 -> Mux/2
  Constant5/1 -> Saturation Dynamic/1
  Saturation/1 -> Mux/1
  T_req/1 -> Saturation Dynamic/2
  Crankshaft_speed/1 -> Product/2
  1-D Lookup Table/1 -> Saturation Dynamic/3
  [speed] -> 1-D Lookup Table/1

== system Porsche930Turbo_Model_V0/ECU/Hybrid_Mode ==
  T_req : Inport
  Crankshaft_speed : Inport  Port=2
  SoC : Inport  Port=3
  " " : Constant  Value=0
  "   " : Constant  Value=tmax_ice
  "    " : simulink/Discontinuities/Saturation Dynamic  OutMin=[]  OutMax=[]  OutDataTypeStr=Inherit: Same as second input  OutDataType=fixdt(1, 16)  OutScaling=2^-10  DoSatur=off
  1-D Lookup Table : Lookup_n-D  NumberOfTableDimensions=1  BreakpointsForDimension1=v_cutoff_bp  Table=-temax_em * v_cutoff_tbl  InternalRulePriority=Speed  RndMeth=Simplest
  MATLAB Function : MATLAB Function  TreatAsAtomicUnit=on
  Mux : Mux  Inputs=2
  Sat_EM : simulink/Discontinuities/Saturation Dynamic  OutMin=[]  OutMax=[]  OutDataTypeStr=Inherit: Same as second input  OutDataType=fixdt(1, 16)  OutScaling=2^-10  DoSatur=off
  Standard1 : Lookup_n-D  NumberOfTableDimensions=1  BreakpointsForDimension1=ne_em  Table=te_em  InternalRulePriority=Speed  RndMeth=Simplest
  to RPM : Gain  Gain=60 / (2 * pi)
  T_actual : Outport
  wires:
  T_req/1 -> MATLAB Function/1(t_req)
  Crankshaft_speed/1 -> to RPM/1
  MATLAB Function/1(t_ICE) -> "    "/2
  "   "/1 -> "    "/1
  " "/1 -> "    "/3
  "    "/1 -> Mux/1  "T_ICE"
  Sat_EM/1 -> Mux/2  "T_EMOT"
  Mux/1 -> T_actual/1
  to RPM/1 -> Standard1/1
  MATLAB Function/2(t_em) -> Sat_EM/2
  [speed] -> 1-D Lookup Table/1
  1-D Lookup Table/1 -> Sat_EM/3
  SoC/1 -> MATLAB Function/3(SoC)
  Standard1/1 -> MATLAB Function/2(t_em_max), Sat_EM/1

== system Porsche930Turbo_Model_V0/ECU/ICE_Mode ==
  T_req : Inport
  " " : Constant  Value=tmax_ice
  "  " : Constant  Value=0
  Constant : Constant  Value=0
  Mux : Mux  Inputs=2
  Saturation Dynamic : simulink/Discontinuities/Saturation Dynamic  OutMin=[]  OutMax=[]  OutDataTypeStr=Inherit: Same as second input  OutDataType=fixdt(1, 16)  OutScaling=2^-10  DoSatur=off
  Scope : Scope  NumInputPorts=2
      settings: ActiveDisplayYMinimum=-1  ActiveDisplayYMaximum=1  DataLoggingVariableName=ScopeData14
  T_actual : Outport
  wires:
  Mux/1 -> T_actual/1
  Constant/1 -> Mux/2  "T_EMOT"
  Saturation Dynamic/1 -> Scope/2, Mux/1  "T_ICE"
  " "/1 -> Saturation Dynamic/1
  "  "/1 -> Saturation Dynamic/3
  T_req/1 -> Scope/1, Saturation Dynamic/2  "PWT_Torque"

== system Porsche930Turbo_Model_V0/ECU/RACE_Mode ==
  T_req : Inport
  Crankshaft_speed : Inport  Port=2
  SoC : Inport  Port=3
  % : simulink/Logic and Bit Operations/Compare To Constant  relop=>=  const=0.3  OutDataTypeStr=boolean
  1-D Lookup Table : Lookup_n-D  NumberOfTableDimensions=1  BreakpointsForDimension1=v_cutoff_bp  Table=-temax_em * v_cutoff_tbl  InternalRulePriority=Speed  RndMeth=Simplest
  AND1 : Logic  Inputs=3  IconShape=distinctive  AllPortsSameDT=off  OutDataTypeStr=boolean
  Constant2 : Constant  Value=tmax_ice
  Mux : Mux  Inputs=2
  Overboost : Lookup_n-D  NumberOfTableDimensions=1  BreakpointsForDimension1=ne_em  Table=te_em_peak  InternalRulePriority=Speed  RndMeth=Simplest
  RPM_Boost : simulink/Logic and Bit Operations/Compare To Constant  relop=<=  const=2800  OutDataTypeStr=boolean
  Req_Boost : simulink/Logic and Bit Operations/Compare To Constant  relop=>=  const=250  OutDataTypeStr=boolean
  Saturation Dynamic : simulink/Discontinuities/Saturation Dynamic  OutMin=[]  OutMax=[]  OutDataTypeStr=Inherit: Same as second input  OutDataType=fixdt(1, 16)  OutScaling=2^-10  DoSatur=off
  Saturation Dynamic1 : simulink/Discontinuities/Saturation Dynamic  OutMin=[]  OutMax=[]  OutDataTypeStr=Inherit: Same as second input  OutDataType=fixdt(1, 16)  OutScaling=2^-10  DoSatur=off
  Standard : Lookup_n-D  NumberOfTableDimensions=1  BreakpointsForDimension1=ne_em  Table=te_em  InternalRulePriority=Speed  RndMeth=Simplest
  Switch2 : Switch  Criteria=u2 > Threshold  SaturateOnIntegerOverflow=off  InputSameDT=off
  idle torque : Constant  Value=0
  to RPM : Gain  Gain=60 / (2 * pi)
  T_actual : Outport
  wires:
  idle torque/1 -> Saturation Dynamic/3
  Mux/1 -> T_actual/1
  Saturation Dynamic/1 -> Mux/1  "T_ICE"
  Saturation Dynamic1/1 -> Mux/2  "T_EMOT"
  1-D Lookup Table/1 -> Saturation Dynamic1/3
  Constant2/1 -> Saturation Dynamic/1
  [speed] -> 1-D Lookup Table/1
  T_req/1 -> Saturation Dynamic/2, Saturation Dynamic1/2, Req_Boost/1
  Standard/1 -> Switch2/3
  Overboost/1 -> Switch2/1
  AND1/1 -> Switch2/2
  to RPM/1 -> Overboost/1, Standard/1, RPM_Boost/1
  Crankshaft_speed/1 -> to RPM/1
  Switch2/1 -> Saturation Dynamic1/1
  SoC/1 -> %/1
  %/1 -> AND1/1
  Req_Boost/1 -> AND1/2
  RPM_Boost/1 -> AND1/3

== system Porsche930Turbo_Model_V0/ICE/ICE energy consumption ==
  RPM : Inport
  T_ICE : Inport  Port=2
  Constant : Constant  Value=0
  Fuel : Gain  Gain=bsfc / (1000 * rho_fuel)
  Fuel [L] : Display
  Gain : Gain  Gain=2.778e-7
  Gain1 : Gain  Gain=pi/30
  Integrator : Integrator
  Joule : Display
  Product : Product
  Switch : Switch  Criteria=u2 > Threshold  SaturateOnIntegerOverflow=off  InputSameDT=off
  To Workspace1 : ToWorkspace  VariableName=P_ICE  SampleTime=-1
  kWh : Display
  P_ICE [W] : Outport
  tag scope: Fuel_Liters=global
  wires:
  RPM/1 -> Gain1/1
  Integrator/1 -> Gain/1, Joule/1
  Gain/1 -> kWh/1, Fuel/1
  Gain1/1 -> Product/2
  Product/1 -> P_ICE [W]/1, To Workspace1/1, Integrator/1
  T_ICE/1 -> Switch/2, Switch/1
  Switch/1 -> Product/1
  Constant/1 -> Switch/3
  Fuel/1 -> [Fuel_Liters], Fuel [L]/1

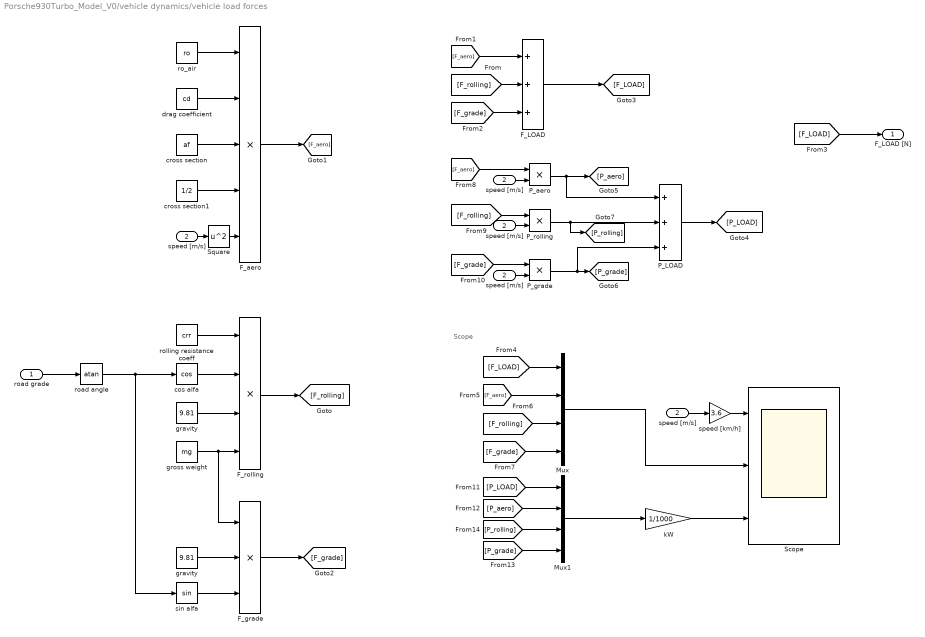
== system Porsche930Turbo_Model_V0/vehicle dynamics/vehicle load forces ==
  note: Scope
  road grade : Inport
  speed [m/s] : Inport  Port=2
  F_LOAD : Sum  Inputs=+++
  F_aero : Product  Inputs=5
  F_grade : Product  Inputs=3
  F_rolling : Product  Inputs=4
  Mux : Mux
  Mux1 : Mux
  P_LOAD : Sum  Inputs=+++
  P_aero : Product
  P_grade : Product
  P_rolling : Product
  Scope : Scope  NumInputPorts=3
      settings: Title=SPEED  ActiveDisplayYMinimum=-1  ActiveDisplayYMaximum=1  DataLoggingSaveFormat=Array
  Square : Math  Operator=square
  cos alfa : Trigonometry  Operator=cos
  cross section : Constant  Value=af
  cross section1 : Constant  Value=1/2
  drag coefficient : Constant  Value=cd
  gravity : Constant  Value=9.81
  "gravity " : Constant  Value=9.81
  gross weight : Constant  Value=mg
  kW : Gain  Gain=1/1000
  ro_air : Constant  Value=ro
  road angle : Trigonometry  Operator=atan
  rolling resistance coeff : Constant  Value=crr
  sin alfa : Trigonometry
  speed [km/h] : Gain  Gain=3.6
  "speed [m/s] " : InportShadow  Port=2
  "speed [m/s]  " : InportShadow  Port=2
  "speed [m/s]   " : InportShadow  Port=2
  "speed [m/s]    " : InportShadow  Port=2
  F_LOAD [N] : Outport
  wires:
  ro_air/1 -> F_aero/1
  drag coefficient/1 -> F_aero/2
  cross section/1 -> F_aero/3
  cross section1/1 -> F_aero/4
  F_aero/1 -> [F_aero]
  road grade/1 -> road angle/1
  road angle/1 -> sin alfa/1, cos alfa/1
  rolling resistance coeff/1 -> F_rolling/1
  cos alfa/1 -> F_rolling/2
  gravity/1 -> F_rolling/3
  gross weight/1 -> F_grade/1, F_rolling/4
  sin alfa/1 -> F_grade/3
  F_LOAD/1 -> [F_LOAD]
  F_rolling/1 -> [F_rolling]
  F_grade/1 -> [F_grade]
  P_aero/1 -> [P_aero], P_LOAD/1
  P_rolling/1 -> [P_rolling], P_LOAD/2
  P_grade/1 -> [P_grade], P_LOAD/3
  speed [km/h]/1 -> Scope/1
  Mux/1 -> Scope/2
  kW/1 -> Scope/3
  "speed [m/s] "/1 -> P_aero/2
  "speed [m/s]  "/1 -> speed [km/h]/1
  "speed [m/s]   "/1 -> P_rolling/2
  "speed [m/s]    "/1 -> P_grade/2
  Square/1 -> F_aero/5
  speed [m/s]/1 -> Square/1
  "gravity "/1 -> F_grade/2
  [F_rolling] -> F_LOAD/2
  [F_aero] -> F_LOAD/1
  [F_grade] -> F_LOAD/3
  [F_LOAD] -> F_LOAD [N]/1
  [F_LOAD] -> Mux/1
  [F_aero] -> Mux/2
  [F_rolling] -> Mux/3
  [F_grade] -> Mux/4
  [F_aero] -> P_aero/1
  [F_rolling] -> P_rolling/1
  [F_grade] -> P_grade/1
  P_LOAD/1 -> [P_LOAD]
  [P_LOAD] -> Mux1/1
  [P_aero] -> Mux1/2
  [P_grade] -> Mux1/4
  [P_rolling] -> Mux1/3
  Mux1/1 -> kW/1

== system Porsche930Turbo_Model_V0/Battery Pack/Subsystem/BMS ==
  vB(t) [V] : Inport
  iB [A] : Inport  Port=2
  CellT [°C] : Inport  Port=3
  Chart : Stateflow chart  TreatAsAtomicUnit=on
  Current1 : Logic  Inputs=3  IconShape=distinctive  AllPortsSameDT=off  OutDataTypeStr=boolean
  IMAX : simulink/Logic and Bit Operations/Compare To Constant  relop=<  const=70  OutDataTypeStr=boolean
  NOT : Logic  Operator=NOT  IconShape=distinctive  AllPortsSameDT=off  OutDataTypeStr=boolean
  Scope : Scope  NumInputPorts=3
      settings: ActiveDisplayYMinimum=-1  ActiveDisplayYMaximum=1  DataLoggingSaveFormat=Array
  Temperature : Logic  IconShape=distinctive  AllPortsSameDT=off  OutDataTypeStr=boolean
  Vmax : simulink/Logic and Bit Operations/Compare To Constant  relop=<  const=425  OutDataTypeStr=boolean
  Vmax2 : simulink/Logic and Bit Operations/Compare To Constant  relop=<  const=60  OutDataTypeStr=boolean
  Vmin : simulink/Logic and Bit Operations/Compare To Constant  relop=>  const=0  OutDataTypeStr=boolean
  Vmin2 : simulink/Logic and Bit Operations/Compare To Constant  relop=>  const=-10  OutDataTypeStr=boolean
  Voltage : Logic  IconShape=distinctive  AllPortsSameDT=off  OutDataTypeStr=boolean
  StopCondition : Outport
  tag scope: StopCondition=global
  wires:
  Vmin/1 -> Voltage/2
  Vmax/1 -> Voltage/1
  IMAX/1 -> Scope/2, Current1/2
  Voltage/1 -> Scope/1, Current1/1
  Temperature/1 -> Scope/3, Current1/3
  Current1/1 -> NOT/1
  vB(t) [V]/1 -> Vmin/1, Vmax/1
  Vmax2/1 -> Temperature/1
  Vmin2/1 -> Temperature/2
  CellT [°C]/1 -> Vmax2/1, Vmin2/1
  iB [A]/1 -> IMAX/1
  NOT/1 -> Chart/1(StopCondition)
  Chart/2(CurrentCondition) -> [StopCondition]
  Chart/1(StopConditionOut) -> StopCondition/1
